simulink model "furuta_urdf_test"  (R2025b)
settings: Solver=VariableStepAuto  StartTime=0.0  StopTime=10.0  RelTol=1e-3
settings Model: Creator=Compu  LastModifiedBy=Compu

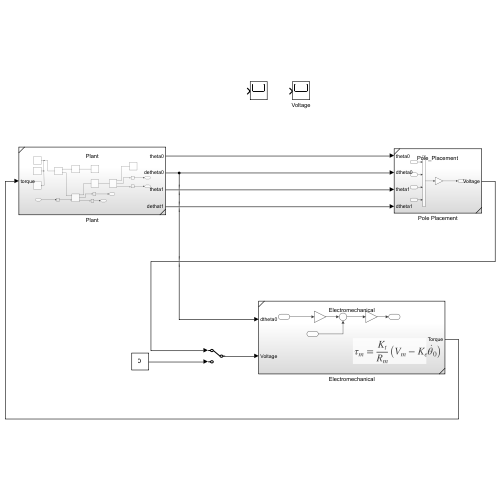
[thumbnail: Simulink's stored preview of the top-level diagram]
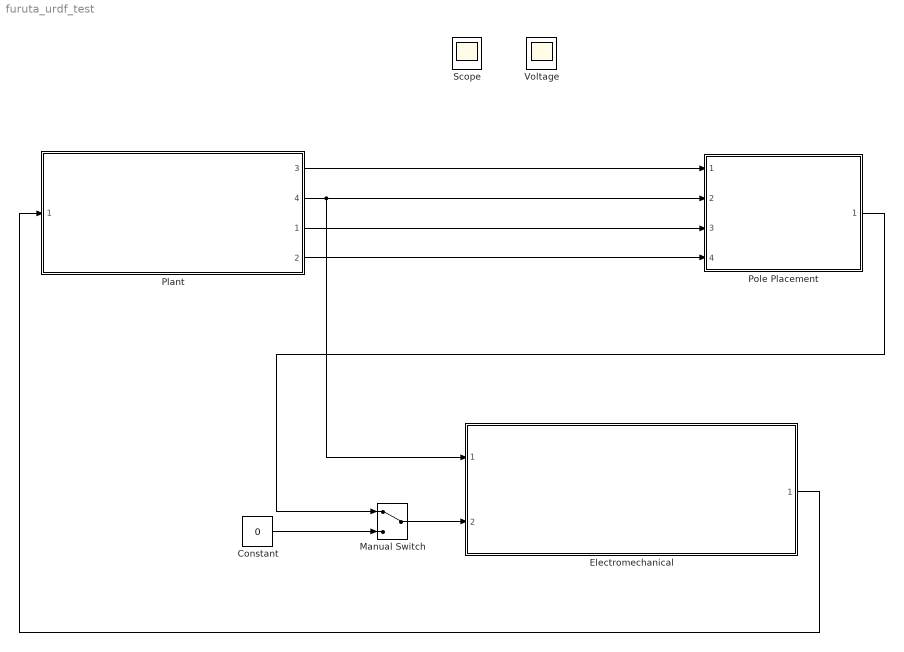
== system furuta_urdf_test ==
  Constant : Constant  Value=0
  Electromechanical : Subsystem  ReferencedSubsystem=Electromechanical
  Manual Switch : ManualSwitch
  Plant : Subsystem  ReferencedSubsystem=Plant
      settings: PortSchema="{\"entries\":[{\"content\":{\"sides\":[{\"content\":{\"connectorIds\":[\"In1\"]},\"type\":\"ConnectorPlacement.EquallySpacedRectSide\",\"uuid\":\"698e2142-6e18-4f9d-97c1-5a83dc679f38\"},{\"content\":{\"connectorIds\":[\"Out3\",\"Out4\",\"Out1\",\"Out2\"],\"side\":\"RIGHT\"},\"type\":\"ConnectorPlacement.EquallySpacedRectSide\",\"uuid\":\"8da0675e-fcb1-4bf9-9de6-c47ad67b018d\"},{\"content\":{\"side\":\"TOP\"},\"type\":\"ConnectorPlacement.EquallySpacedRectSide\",\"uuid\":\"bb61f6dc-b80a-4d58-a0df-5270abb20313\"}]},\"type\":\"ConnectorPlacement.EquallySpacedConnector\",\"uuid\":\"677f761d-6bde-4c02-9291-1daa9ae2b3af\"}],\"packageUris\":[\"http://schema.mathworks.com/mf0/Connector/R2020b\"],\"version\":\"1.0\"}"
  Pole Placement : Subsystem  ReferencedSubsystem=Pole_Placement
  Scope : Scope
  Voltage : Scope
      settings: ActiveDisplayYMinimum=-3.2199569205274443  ActiveDisplayYMaximum=0.60844546471572569  DataLoggingVariableName=ScopeData4
  wires:
  Plant/4 -> Pole Placement/2, Electromechanical/1
  Electromechanical/1 -> Plant/1
  Plant/3 -> Pole Placement/1
  Plant/1 -> Pole Placement/3
  Plant/2 -> Pole Placement/4
  Manual Switch/1 -> Electromechanical/2
  Constant/1 -> Manual Switch/2
  Pole Placement/1 -> Manual Switch/1
